simulink model "pid_anti_windup_clamping_ver1"  (R2026b)
settings: Solver=ode4  StopTime=30  FixedStep=0.05
settings Model: Creator=ZAID  LastModifiedBy=ZAID

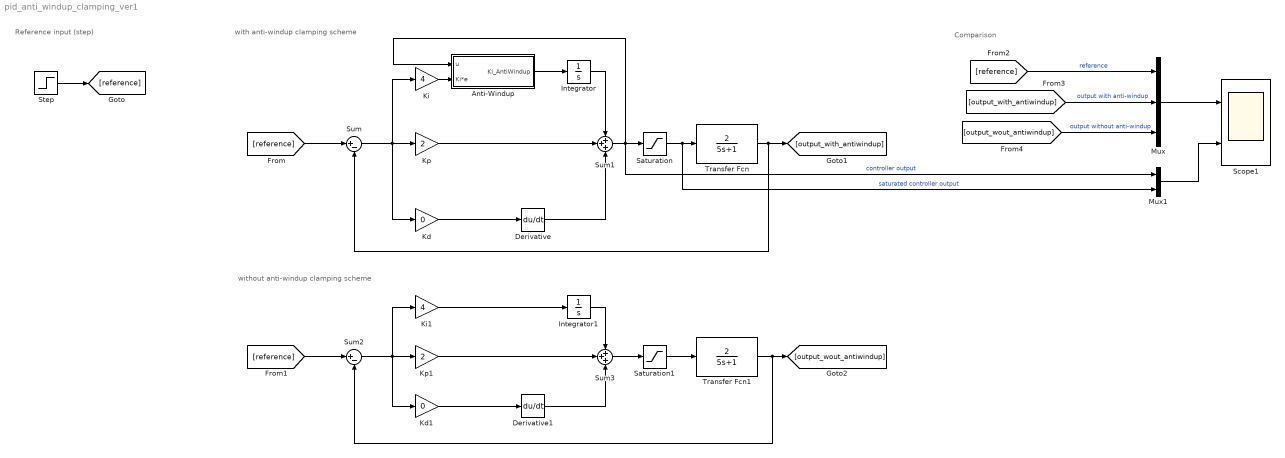
== system pid_anti_windup_clamping_ver1 ==
  note: Comparison
  note: Reference input (step)
  note: with anti-windup clamping scheme
  note: without anti-windup clamping scheme
  Anti-Windup : Subsystem
  Derivative : Derivative
  Derivative1 : Derivative
  Integrator : Integrator
  Integrator1 : Integrator
  Kd : Gain  Gain=0
  Kd1 : Gain  Gain=0
  Ki : Gain  Gain=4
  Ki1 : Gain  Gain=4
  Kp : Gain  Gain=2
  Kp1 : Gain  Gain=2
  Mux : Mux  Inputs=3
  Mux1 : Mux  Inputs=2
  Saturation : Saturate  UpperLimit=10  LowerLimit=-10
      settings: AttributesFormatString=|
      | u_max = %<UpperLimit>
      | u_min = %<LowerLimit>
  Saturation1 : Saturate  UpperLimit=10  LowerLimit=-10
      settings: AttributesFormatString=|
      | u_max = %<UpperLimit>
      | u_min = %<LowerLimit>
  Scope1 : Scope  NumInputPorts=2
      settings: ActiveDisplayYMinimum=-2.4389081814821214  ActiveDisplayYMaximum=21.950173633339098
  Step : Step  FinalValue=15  SampleTime=0
  Sum : Sum  Inputs=|+-
  Sum1 : Sum  Inputs=+++
  Sum2 : Sum  Inputs=|+-
  Sum3 : Sum  Inputs=+++
  Transfer Fcn : TransferFcn  Numerator=2  Denominator=[5 1]
  Transfer Fcn1 : TransferFcn  Numerator=2  Denominator=[5 1]
  wires:
  Sum/1 -> Ki/1, Kd/1, Kp/1
  Kd/1 -> Derivative/1
  Kp/1 -> Sum1/2
  Integrator/1 -> Sum1/1
  Derivative/1 -> Sum1/3
  Sum1/1 -> Anti-Windup/1(u), Mux1/1, Saturation/1  "controller output"
  Transfer Fcn/1 -> [output_with_antiwindup], Sum/2
  Saturation/1 -> Mux1/2, Transfer Fcn/1  "saturated controller output"
  Anti-Windup/1(Ki_AntiWindup) -> Integrator/1
  Ki/1 -> Anti-Windup/2(Ki*e)
  Ki1/1 -> Integrator1/1
  Saturation1/1 -> Transfer Fcn1/1
  Transfer Fcn1/1 -> Sum2/2, [output_wout_antiwindup]
  Sum3/1 -> Saturation1/1
  Derivative1/1 -> Sum3/3
  Integrator1/1 -> Sum3/1
  Kp1/1 -> Sum3/2
  Kd1/1 -> Derivative1/1
  Sum2/1 -> Kp1/1, Kd1/1, Ki1/1
  Step/1 -> [reference]
  [reference] -> Sum/1
  [reference] -> Sum2/1
  [reference] -> Mux/1  "reference"
  [output_with_antiwindup] -> Mux/2  "output with anti-windup"
  [output_wout_antiwindup] -> Mux/3  "output without anti-windup"
  Mux/1 -> Scope1/1
  Mux1/1 -> Scope1/2

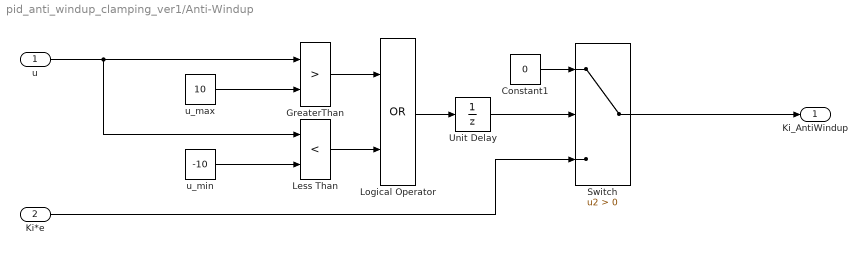
== system pid_anti_windup_clamping_ver1/Anti-Windup ==
  u : Inport
  Ki*e : Inport  Port=2
  Constant1 : Constant  Value=0
  GreaterThan : RelationalOperator  Operator=>  OutDataTypeStr=boolean  RndMeth=Simplest  InputSameDT=off
  Less Than : RelationalOperator  Operator=<  OutDataTypeStr=boolean  RndMeth=Simplest  InputSameDT=off
  Logical Operator : Logic  Operator=OR  AllPortsSameDT=off  OutDataTypeStr=boolean
  Switch : Switch  Criteria=u2 > Threshold  SaturateOnIntegerOverflow=off  InputSameDT=off
  Unit Delay : UnitDelay  SampleTime=-1
  u_max : Constant  Value=10
  u_min : Constant  Value=-10
  Ki_AntiWindup : Outport
  wires:
  u/1 -> Less Than/1, GreaterThan/1
  Ki*e/1 -> Switch/3
  GreaterThan/1 -> Logical Operator/1
  Switch/1 -> Ki_AntiWindup/1
  u_min/1 -> Less Than/2
  u_max/1 -> GreaterThan/2
  Logical Operator/1 -> Unit Delay/1
  Less Than/1 -> Logical Operator/2
  Constant1/1 -> Switch/1
  Unit Delay/1 -> Switch/2
